simulink model "Shaddad_NavFusion"  (R2026b)
undefined symbols (not defined in the file): P, Ts
libraries: simulink x18, robotcorelib x4, ros2lib x3, mspfiltlib x2
(part 1 of 2)
settings Model: Creator=aomar  LastModifiedBy=aomar

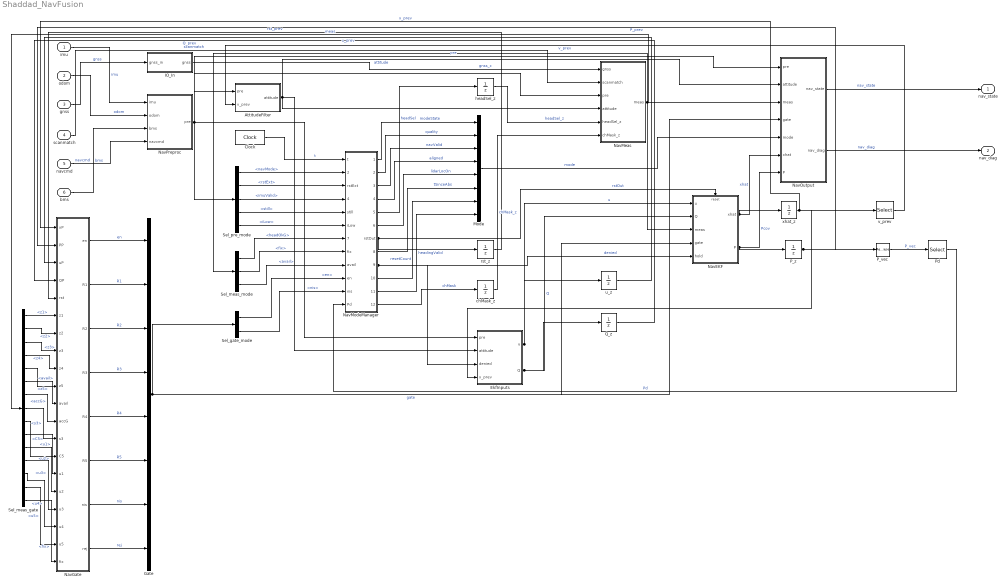
== system Shaddad_NavFusion ==
  imu : Inport  OutDataTypeStr=Bus: Bus_ImuMeas  SampleTime=Ts.imu  BusOutputAsStruct=on
  odom : Inport  Port=2  OutDataTypeStr=Bus: Bus_OdomMeas  SampleTime=Ts.ctrl  BusOutputAsStruct=on
  gnss : Inport  Port=3  OutDataTypeStr=Bus: Bus_GnssRaw  SampleTime=Ts.hk  BusOutputAsStruct=on
  scanmatch : Inport  Port=4  OutDataTypeStr=Bus: Bus_ScanMatchMeas  SampleTime=Ts.gnc_status  BusOutputAsStruct=on
  navcmd : Inport  Port=5  OutDataTypeStr=Bus: Bus_NavCmd  SampleTime=Ts.comm  BusOutputAsStruct=on
  bms : Inport  Port=6  OutDataTypeStr=Bus: Bus_BmsStatus  SampleTime=Ts.hk  BusOutputAsStruct=on
  AttitudeFilter : Subsystem
  Clock : DigitalClock  SampleTime=Ts.nav
  EkfInputs : Subsystem
  Gate : BusCreator  Inputs=8
  IO_In : Subsystem  Variant=on
  Mode : BusCreator  Inputs=8
  NavEKF : Subsystem  Description=EKF (MATLAB System sens_nav_ekf = extendedKalmanFilter, predict + 5 gated corrections at 0.01 s) inside a Resettable Subsystem: navReset rising edge / FAULT re-initialise x0 / P0 (T-NAV-09).  TreatAsAtomicUnit=on
  NavGate : MATLAB Function  TreatAsAtomicUnit=on  mask{prm=P.sensors.navgate}
  NavMeas : Subsystem
  NavModeManager : MATLAB Function  TreatAsAtomicUnit=on  mask{prm=P.sensors.navmode}
  NavOutput : Subsystem
  NavPreproc : Subsystem
  P_vec : Reshape
  P_z : UnitDelay  InitialCondition=P.sensors.ekf.P0  SampleTime=Ts.nav
  Pd : Selector  InputPortWidth=121  IndexOptions=Index vector (dialog)  Indices=[1 13 37]  OutputSizes=1
  Q_z : UnitDelay  InitialCondition=P.sensors.ekf.Qd  SampleTime=Ts.nav
  Sel_gate_mode : BusSelector  OutputSignals=en,nis
  Sel_meas_gate : BusSelector  OutputSignals=z1,z2,z3,z4,z5,avail,accG,s3,C5,u1,u2,u3,u4,u5,fix
  Sel_meas_mode : BusSelector  OutputSignals=headOkG,fix,avail
  Sel_pre_mode : BusSelector  OutputSignals=navMode,rstExt,imuValid,still,iLow
  chMask_z : UnitDelay  InitialCondition=true(5, 1)  SampleTime=Ts.nav
  headSel_z : UnitDelay  SampleTime=Ts.nav
  rst_z : UnitDelay  InitialCondition=false  SampleTime=Ts.nav
  u_z : UnitDelay  InitialCondition=P.sensors.ekf.u0  SampleTime=Ts.nav
  v_prev : Selector  InputPortWidth=11  IndexOptions=Index vector (dialog)  Indices=5  OutputSizes=1
  xhat_z : UnitDelay  InitialCondition=P.sensors.ekf.x0  SampleTime=Ts.nav
  nav_state : Outport  OutDataTypeStr=Bus: Bus_NavState  SampleTime=Ts.ctrl  BusOutputAsStruct=on
  nav_diag : Outport  Port=2  OutDataTypeStr=Bus: Bus_NavDiag  SampleTime=Ts.ctrl  BusOutputAsStruct=on
  wires:
  Sel_meas_gate/1 -> NavGate/6(z1)  "<z1>"
  Sel_meas_gate/2 -> NavGate/7(z2)  "<z2>"
  Sel_meas_gate/3 -> NavGate/8(z3)  "<z3>"
  Sel_meas_gate/4 -> NavGate/9(z4)  "<z4>"
  Sel_meas_gate/5 -> NavGate/10(z5)  "<z5>"
  Sel_meas_gate/6 -> NavGate/11(avail)  "<avail>"
  Sel_meas_gate/8 -> NavGate/13(s3)  "<s3>"
  Sel_meas_gate/10 -> NavGate/15(u1)  "<u1>"
  Sel_meas_gate/12 -> NavGate/17(u3)  "<u3>"
  Sel_meas_gate/14 -> NavGate/19(u5)  "<u5>"
  Sel_meas_gate/15 -> NavGate/20(fix)  "<fix>"
  imu/1 -> NavPreproc/1(imu)  "imu"
  odom/1 -> NavPreproc/2(odom)  "odom"
  gnss/1 -> IO_In/1(gnss_in)  "gnss"
  scanmatch/1 -> NavMeas/2(scanmatch)  "scanmatch"
  navcmd/1 -> NavPreproc/4(navcmd)  "navcmd"
  bms/1 -> NavPreproc/3(bms)  "bms"
  NavGate/1(en) -> Gate/1  "en"
  NavGate/2(R1) -> Gate/2  "R1"
  NavGate/3(R2) -> Gate/3  "R2"
  NavGate/4(R3) -> Gate/4  "R3"
  NavGate/5(R4) -> Gate/5  "R4"
  NavGate/6(R5) -> Gate/6  "R5"
  NavGate/7(nis) -> Gate/7  "nis"
  NavGate/8(rej) -> Gate/8  "rej"
  Gate/1 -> NavOutput/4(gate), NavEKF/4(gate), Sel_gate_mode/1  "gate"
  IO_In/1(gnss) -> NavMeas/1(gnss)  "gnss_c"
  NavPreproc/1(pre) -> EkfInputs/1(pre), Sel_pre_mode/1, NavOutput/1(pre), AttitudeFilter/1(pre), NavMeas/3(pre)  "pre"
  Sel_pre_mode/1 -> NavModeManager/2(navMode)  "<navMode>"
  Sel_pre_mode/2 -> NavModeManager/3(rstExt)  "<rstExt>"
  Sel_pre_mode/3 -> NavModeManager/4(imuValid)  "<imuValid>"
  Sel_pre_mode/4 -> NavModeManager/5(still)  "<still>"
  Sel_pre_mode/5 -> NavModeManager/6(iLow)  "<iLow>"
  Sel_meas_mode/1 -> NavModeManager/7(headOkG)  "<headOkG>"
  Sel_meas_mode/2 -> NavModeManager/8(fix)  "<fix>"
  Sel_meas_mode/3 -> NavModeManager/9(avail)  "<avail>"
  Sel_gate_mode/1 -> NavModeManager/10(en)  "<en>"
  Sel_gate_mode/2 -> NavModeManager/11(nis)  "<nis>"
  Clock/1 -> NavModeManager/1(t)  "t"
  AttitudeFilter/1(attitude) -> EkfInputs/2(attitude), NavOutput/2(attitude), NavMeas/4(attitude)  "attitude"
  NavModeManager/1(modeState) -> Mode/1  "modeState"
  NavModeManager/2(quality) -> Mode/2  "quality"
  NavModeManager/3(navValid) -> Mode/3  "navValid"
  NavModeManager/4(aligned) -> Mode/4  "aligned"
  NavModeManager/5(headSel) -> headSel_z/1  "headSel"
  NavModeManager/6(lidarLocOn) -> Mode/5  "lidarLocOn"
  NavModeManager/7(rstOut) -> NavEKF/Reset, rst_z/1  "rstOut"
  NavModeManager/8(tSinceAbs) -> Mode/6  "tSinceAbs"
  NavModeManager/9(denied) -> EkfInputs/3(denied), NavEKF/5(hold)  "denied"
  NavModeManager/10(resetCount) -> Mode/7  "resetCount"
  NavModeManager/11(headingValid) -> Mode/8  "headingValid"
  NavModeManager/12(chMask) -> chMask_z/1  "chMask"
  Mode/1 -> NavOutput/5(mode)  "mode"
  headSel_z/1 -> NavMeas/5(headSel_z)  "headSel_z"
  rst_z/1 -> NavGate/5(rst)  "rst_prev"
  chMask_z/1 -> NavMeas/6(chMask_z)  "chMask_z"
  EkfInputs/1(u) -> NavEKF/1(u), u_z/1  "u"
  EkfInputs/2(Q) -> NavEKF/2(Q), Q_z/1  "Q"
  u_z/1 -> NavGate/3(uP)  "u_prev"
  NavEKF/1(xhat) -> NavOutput/6(xhat), xhat_z/1  "xhat"
  NavEKF/2(P) -> NavOutput/7(P), P_z/1  "Pcov"
  xhat_z/1 -> EkfInputs/4(x_prev), NavGate/1(xP), v_prev/1  "x_prev"
  P_z/1 -> NavGate/2(PP), P_vec/1  "P_prev"
  NavOutput/1(nav_state) -> nav_state/1  "nav_state"
  NavOutput/2(nav_diag) -> nav_diag/1  "nav_diag"
  P_vec/1 -> Pd/1  "P_vec"
  v_prev/1 -> AttitudeFilter/2(v_prev)  "v_prev"
  Pd/1 -> NavModeManager/12(Pd)  "Pd"
  Q_z/1 -> NavGate/4(QP)  "Q_prev"
  NavMeas/1(meas) -> Sel_meas_gate/1, Sel_meas_mode/1, NavEKF/3(meas), NavOutput/3(meas)  "meas"
  Sel_meas_gate/11 -> NavGate/16(u2)  "<u2>"
  Sel_meas_gate/13 -> NavGate/18(u4)  "<u4>"
  Sel_meas_gate/7 -> NavGate/12(accG)  "<accG>"
  Sel_meas_gate/9 -> NavGate/14(C5)  "<C5>"

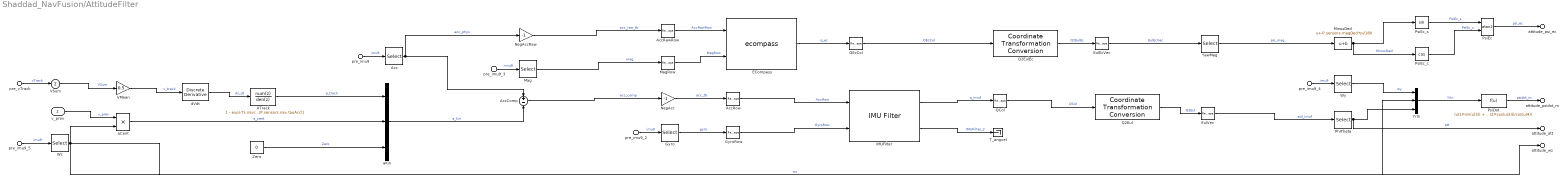
== system Shaddad_NavFusion/AttitudeFilter ==
  pre_imu9 : Inport  PortName=pre  Element=imu9
  pre_imu9_{2..5} (4 alike) : Inport  PortName=pre  Element=imu9
  pre_vTrack : Inport  PortName=pre  Element=vTrack
  v_prev : Inport  Port=2
  ATrack : DiscreteTransferFcn  Numerator=1 - exp(-Ts.nav/P.sensors.nav.tauAcc)  Denominator=[1 -exp(-Ts.nav/P.sensors.nav.tauAcc)]  SampleTime=Ts.nav
  Acc : Selector  InputPortWidth=9  IndexOptions=Index vector (dialog)  Indices=1:3  OutputSizes=1
  AccComp : Sum  Inputs=+-
  AccRawRow : Reshape  OutputDimensionality=Customize  OutputDimensions=[1 3]
  AccRow : Reshape  OutputDimensionality=Customize  OutputDimensions=[1 3]
  ECompass : mspfiltlib/ecompass  ReferenceFrame=ENU  OrientationFormat=quaternion  SimulateUsing=Code generation
  EulEcVec : Reshape
  EulVec : Reshape
  Gyro : Selector  InputPortWidth=9  IndexOptions=Index vector (dialog)  Indices=4:6  OutputSizes=1
  GyroRow : Reshape  OutputDimensionality=Customize  OutputDimensions=[1 3]
  IMUFilter : mspfiltlib/IMU Filter  DispRefFrame=ENU  OrientationFormat=quaternion  DecimationFactor=1  InitialProcessNoise=P.sensors.nav.imufQ0  AccelerometerNoise=P.sensors.imuf.AccelerometerNoise  GyroscopeNoise=P.sensors.imuf.GyroscopeNoise  GyroscopeDriftNoise=P.sensors.imuf.GyroscopeDriftNoise  LinearAccelerationNoise=P.sensors.imuf.LinearAccelerationNoise  LinearAccelerationDecayFactor=P.sensors.imuf.LinearAccelerationDecayFactor  SimulateUsing=Code generation
  Mag : Selector  InputPortWidth=9  IndexOptions=Index vector (dialog)  Indices=7:9  OutputSizes=1
  MagRow : Reshape  OutputDimensionality=Customize  OutputDimensions=[1 3]
  MinusDecl : Bias  Bias=-P.sensors.magDecl*pi/180  SaturateOnIntegerOverflow=off
  NegAcc : Gain  Gain=-1
  NegAccRaw : Gain  Gain=-1
  PhiTheta : Selector  InputPortWidth=3  IndexOptions=Index vector (dialog)  Indices=[3 2]  OutputSizes=1
  PsiDot : Fcn  Expr=(u(1)*sin(u(3)) + u(2)*cos(u(3)))/cos(u(4))
  PsiEc : Trigonometry  Operator=atan2
  PsiEc_c : Trigonometry  Operator=cos
  PsiEc_s : Trigonometry
  Q2Eul : robotcorelib/Coordinate Transformation Conversion  InputRepresentation=Quaternion  InputEulerSequence=ZYX  ShowTrVecInputPort=on  OutputRepresentation=Euler Angles  OutputEulerSequence=ZYX  ShowTrVecOutputPort=on  SimulateUsing=Interpreted execution
      settings: LibrarySourceBlock=navlib/Utilities/Coordinate Transformation Conversion
  Q2EulEc : robotcorelib/Coordinate Transformation Conversion  InputRepresentation=Quaternion  InputEulerSequence=ZYX  ShowTrVecInputPort=on  OutputRepresentation=Euler Angles  OutputEulerSequence=ZYX  ShowTrVecOutputPort=on  SimulateUsing=Interpreted execution
      settings: LibrarySourceBlock=navlib/Utilities/Coordinate Transformation Conversion
  QCol : Reshape  OutputDimensionality=Column vector (2-D)
  QEcCol : Reshape  OutputDimensionality=Column vector (2-D)
  T_angvel : Terminator
  VMean : Gain  Gain=0.5
  VSum : Sum  Inputs=+
  Wy : Selector  InputPortWidth=9  IndexOptions=Index vector (dialog)  Indices=5  OutputSizes=1
  Wz : Selector  InputPortWidth=9  IndexOptions=Index vector (dialog)  Indices=6  OutputSizes=1
  YawMag : Selector  InputPortWidth=3  IndexOptions=Index vector (dialog)  Indices=1  OutputSizes=1
  YrIn : Concatenate  NumInputs=3
  Zero : Constant  Value=0
  aCent : Product
  aKin : Concatenate  NumInputs=3
  dVdt : simulink/Discrete/Discrete Derivative  gainval=1  ICPrevScaledInput=0  OutMin=[]  OutMax=[]  OutDataType=fixdt(1, 16)  OutScaling=2^-10  DoSatur=off
  attitude_att : Outport  PortName=attitude  Element=att
  attitude_psi_ec : Outport  PortName=attitude  Element=psi_ec
  attitude_psidot_m : Outport  PortName=attitude  Element=psidot_m
  attitude_wz : Outport  PortName=attitude  Element=wz
  wires:
  pre_vTrack/1 -> VSum/1  "vTrack"
  pre_imu9_5/1 -> Wz/1  "imu9"
  VSum/1 -> VMean/1  "VSum"
  v_prev/1 -> aCent/1  "v_prev"
  Wz/1 -> YrIn/2, aCent/2, attitude_wz/1  "wz"
  VMean/1 -> dVdt/1  "v_track"
  aCent/1 -> aKin/2  "a_cent"
  dVdt/1 -> ATrack/1  "dv_dt"
  Zero/1 -> aKin/3  "Zero"
  ATrack/1 -> aKin/1  "a_track"
  pre_imu9/1 -> Acc/1  "imu9"
  aKin/1 -> AccComp/2  "a_kin"
  Acc/1 -> AccComp/1, NegAccRaw/1  "acc_phys"
  pre_imu9_3/1 -> Mag/1  "imu9"
  AccComp/1 -> NegAcc/1  "acc_comp"
  NegAccRaw/1 -> AccRawRow/1  "acc_raw_tb"
  Mag/1 -> MagRow/1  "mag"
  pre_imu9_2/1 -> Gyro/1  "imu9"
  AccRawRow/1 -> ECompass/1  "AccRawRow"
  MagRow/1 -> ECompass/2  "MagRow"
  NegAcc/1 -> AccRow/1  "acc_tb"
  Gyro/1 -> GyroRow/1  "gyro"
  AccRow/1 -> IMUFilter/1  "AccRow"
  GyroRow/1 -> IMUFilter/2  "GyroRow"
  ECompass/1 -> QEcCol/1  "q_ec"
  QEcCol/1 -> Q2EulEc/1  "QEcCol"
  IMUFilter/1 -> QCol/1  "q_imuf"
  IMUFilter/2 -> T_angvel/1  "IMUFilter_2"
  QCol/1 -> Q2Eul/1  "QCol"
  Q2EulEc/1 -> EulEcVec/1  "Q2EulEc"
  EulEcVec/1 -> YawMag/1  "EulEcVec"
  Q2Eul/1 -> EulVec/1  "Q2Eul"
  EulVec/1 -> PhiTheta/1  "eul_imuf"
  YawMag/1 -> MinusDecl/1  "psi_mag"
  pre_imu9_4/1 -> Wy/1  "imu9"
  MinusDecl/1 -> PsiEc_s/1, PsiEc_c/1  "MinusDecl"
  Wy/1 -> YrIn/1  "wy"
  PhiTheta/1 -> YrIn/3, attitude_att/1  "att"
  YrIn/1 -> PsiDot/1  "YrIn"
  PsiEc_s/1 -> PsiEc/1  "PsiEc_s"
  PsiEc_c/1 -> PsiEc/2  "PsiEc_c"
  PsiEc/1 -> attitude_psi_ec/1  "psi_ec"
  PsiDot/1 -> attitude_psidot_m/1  "psidot_m"

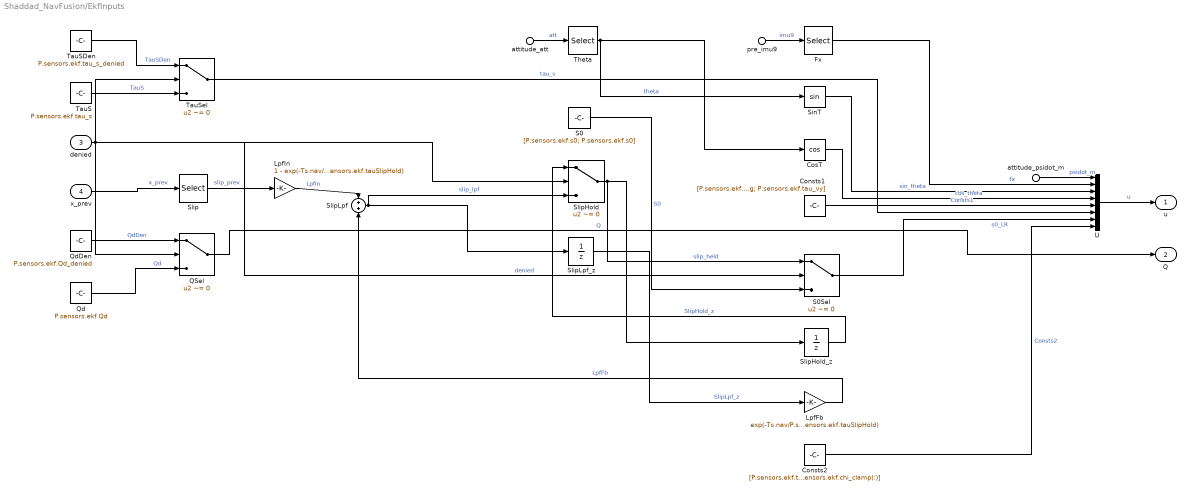
== system Shaddad_NavFusion/EkfInputs ==
  pre_imu9 : Inport  PortName=pre  Element=imu9
  attitude_att : Inport  Port=2  PortName=attitude  Element=att
  attitude_psidot_m : Inport  Port=2  PortName=attitude  Element=psidot_m
  denied : Inport  Port=3
  x_prev : Inport  Port=4
  Consts1 : Constant  Value=[P.sensors.ekf.Ts; P.sensors.g; P.sensors.ekf.tau_vy]
  Consts2 : Constant  Value=[P.sensors.ekf.tau_chi; P.sensors.ekf.chi0; P.sensors.ekf.slip_clamp(:); P.sensors.ekf.chi_clamp(:)]
  CosT : Trigonometry  Operator=cos
  Fx : Selector  InputPortWidth=9  IndexOptions=Index vector (dialog)  Indices=1  OutputSizes=1
  LpfFb : Gain  Gain=exp(-Ts.nav/P.sensors.ekf.tauSlipHold)
  LpfIn : Gain  Gain=1 - exp(-Ts.nav/P.sensors.ekf.tauSlipHold)
  QSel : Switch  Criteria=u2 ~= 0  SaturateOnIntegerOverflow=off  InputSameDT=off
  Qd : Constant  Value=P.sensors.ekf.Qd
  QdDen : Constant  Value=P.sensors.ekf.Qd_denied
  S0 : Constant  Value=[P.sensors.ekf.s0; P.sensors.ekf.s0]
  S0Sel : Switch  Criteria=u2 ~= 0  SaturateOnIntegerOverflow=off  InputSameDT=off
  SinT : Trigonometry
  Slip : Selector  InputPortWidth=11  IndexOptions=Index vector (dialog)  Indices=9:10  OutputSizes=1
  SlipHold : Switch  Criteria=u2 ~= 0  SaturateOnIntegerOverflow=off  InputSameDT=off
  SlipHold_z : UnitDelay  InitialCondition=[P.sensors.ekf.s0; P.sensors.ekf.s0]  SampleTime=Ts.nav
  SlipLpf : Sum
  SlipLpf_z : UnitDelay  InitialCondition=[P.sensors.ekf.s0; P.sensors.ekf.s0]  SampleTime=Ts.nav
  TauS : Constant  Value=P.sensors.ekf.tau_s
  TauSDen : Constant  Value=P.sensors.ekf.tau_s_denied
  TauSel : Switch  Criteria=u2 ~= 0  SaturateOnIntegerOverflow=off  InputSameDT=off
  Theta : Selector  InputPortWidth=2  IndexOptions=Index vector (dialog)  Indices=2  OutputSizes=1
  U : Concatenate  NumInputs=8
  u : Outport
  Q : Outport  Port=2
  wires:
  TauSDen/1 -> TauSel/1  "TauSDen"
  TauS/1 -> TauSel/3  "TauS"
  denied/1 -> S0Sel/2, QSel/2, TauSel/2, SlipHold/2  "denied"
  x_prev/1 -> Slip/1  "x_prev"
  QdDen/1 -> QSel/1  "QdDen"
  Qd/1 -> QSel/3  "Qd"
  Slip/1 -> LpfIn/1  "slip_prev"
  TauSel/1 -> U/6  "tau_s"
  QSel/1 -> Q/1  "Q"
  LpfIn/1 -> SlipLpf/1  "LpfIn"
  SlipLpf/1 -> SlipLpf_z/1, SlipHold/3  "slip_lpf"
  attitude_att/1 -> Theta/1  "att"
  S0/1 -> S0Sel/3  "S0"
  SlipLpf_z/1 -> LpfFb/1  "SlipLpf_z"
  Theta/1 -> CosT/1, SinT/1  "theta"
  SlipHold/1 -> SlipHold_z/1, S0Sel/1  "slip_held"
  pre_imu9/1 -> Fx/1  "imu9"
  SinT/1 -> U/3  "sin_theta"
  CosT/1 -> U/4  "cos_theta"
  Consts1/1 -> U/5  "Consts1"
  LpfFb/1 -> SlipLpf/2  "LpfFb"
  Consts2/1 -> U/8  "Consts2"
  SlipHold_z/1 -> SlipHold/1  "SlipHold_z"
  Fx/1 -> U/2  "fx"
  S0Sel/1 -> U/7  "s0_LR"
  attitude_psidot_m/1 -> U/1  "psidot_m"
  U/1 -> u/1  "u"

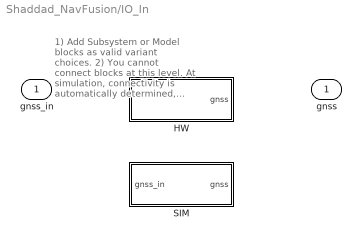
== system Shaddad_NavFusion/IO_In ==
  note: 1) Add Subsystem or Model blocks as valid variant choices.
      | 2) You cannot connect blocks at this level. At simulation, connectivity is automatically
      | determined, based on the active variant and port name matching.
  gnss_in : Inport
  HW : Subsystem  Description=sens_acq_gnss (T12, HW choice of Shaddad_NavFusion/IO_In, VC_TARGET == 1; 0.1 s). Ports: out 1 gnss Bus_GnssRaw 0.1. ros2lib/Subscribe (At sample time) of the ROS 2 ublox driver standard topics: /fix sensor_msgs/NavSatFix (t_meas = header.stamp, lla, hAcc / vAcc = sqrt(position_covariance(1 / 9)), fixType from status: -1 -> 0, 0 / 1 -> 1, 2 -> 4 if hAcc < rtkFixedAcc else 5; newData = IsNew), /fix_velocity geometry_msgs/TwistWithCovarianceStamped (vel_ENU, sAcc), /navheading sensor_msgs/Imu (baseline yaw ENU -> heading_deg = mod(90 - yaw, 360), headAcc_deg, headingValid = IsNew and headAcc < headAccMax_deg). numSV and corrAge are not carried by the standard messages (0). Parameters P.sensors.acq_gnss.  VariantControl=VC_TARGET == 1
  SIM : Subsystem  VariantControl=VC_TARGET == 0
  gnss : Outport

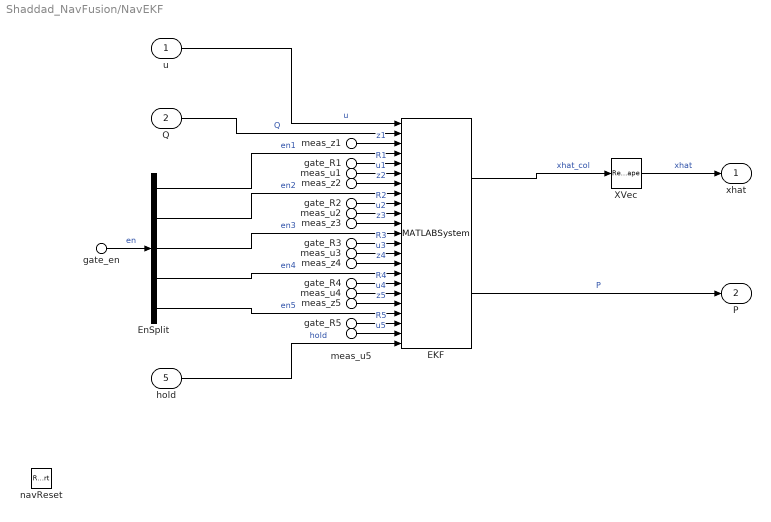
== system Shaddad_NavFusion/NavEKF ==
  u : Inport
  Q : Inport  Port=2
  meas_z1 : Inport  Port=3  PortName=meas  Element=z1
  meas_u1 : Inport  Port=3  PortName=meas  Element=u1
  meas_z2 : Inport  Port=3  PortName=meas  Element=z2
  meas_u2 : Inport  Port=3  PortName=meas  Element=u2
  meas_z3 : Inport  Port=3  PortName=meas  Element=z3
  meas_u3 : Inport  Port=3  PortName=meas  Element=u3
  meas_z4 : Inport  Port=3  PortName=meas  Element=z4
  meas_u4 : Inport  Port=3  PortName=meas  Element=u4
  meas_z5 : Inport  Port=3  PortName=meas  Element=z5
  meas_u5 : Inport  Port=3  PortName=meas  Element=u5
  gate_en : Inport  Port=4  PortName=gate  Element=en
  gate_R1 : Inport  Port=4  PortName=gate  Element=R1
  gate_R2 : Inport  Port=4  PortName=gate  Element=R2
  gate_R3 : Inport  Port=4  PortName=gate  Element=R3
  gate_R4 : Inport  Port=4  PortName=gate  Element=R4
  gate_R5 : Inport  Port=4  PortName=gate  Element=R5
  hold : Inport  Port=5
  navReset : ResetPort  DisableCoverage=on
  EKF : MATLABSystem  System=sens_nav_ekf  InitialState=P.sensors.ekf.x0  InitialStateCovariance=P.sensors.ekf.P0
      mask Type: sens_nav_ekf
  EnSplit : Demux  Outputs=5
  XVec : Reshape
  xhat : Outport
  P : Outport  Port=2
  wires:
  gate_en/1 -> EnSplit/1  "en"
  EnSplit/1 -> EKF/4  "en1"
  EnSplit/2 -> EKF/8  "en2"
  EnSplit/3 -> EKF/12  "en3"
  EnSplit/4 -> EKF/16  "en4"
  EnSplit/5 -> EKF/20  "en5"
  u/1 -> EKF/1  "u"
  Q/1 -> EKF/2  "Q"
  hold/1 -> EKF/23  "hold"
  meas_z1/1 -> EKF/3  "z1"
  gate_R1/1 -> EKF/5  "R1"
  meas_u1/1 -> EKF/6  "u1"
  meas_z2/1 -> EKF/7  "z2"
  gate_R2/1 -> EKF/9  "R2"
  meas_u2/1 -> EKF/10  "u2"
  meas_z3/1 -> EKF/11  "z3"
  gate_R3/1 -> EKF/13  "R3"
  meas_u3/1 -> EKF/14  "u3"
  meas_z4/1 -> EKF/15  "z4"
  gate_R4/1 -> EKF/17  "R4"
  meas_u4/1 -> EKF/18  "u4"
  meas_z5/1 -> EKF/19  "z5"
  gate_R5/1 -> EKF/21  "R5"
  meas_u5/1 -> EKF/22  "u5"
  EKF/1 -> XVec/1  "xhat_col"
  EKF/2 -> P/1  "P"
  XVec/1 -> xhat/1  "xhat"

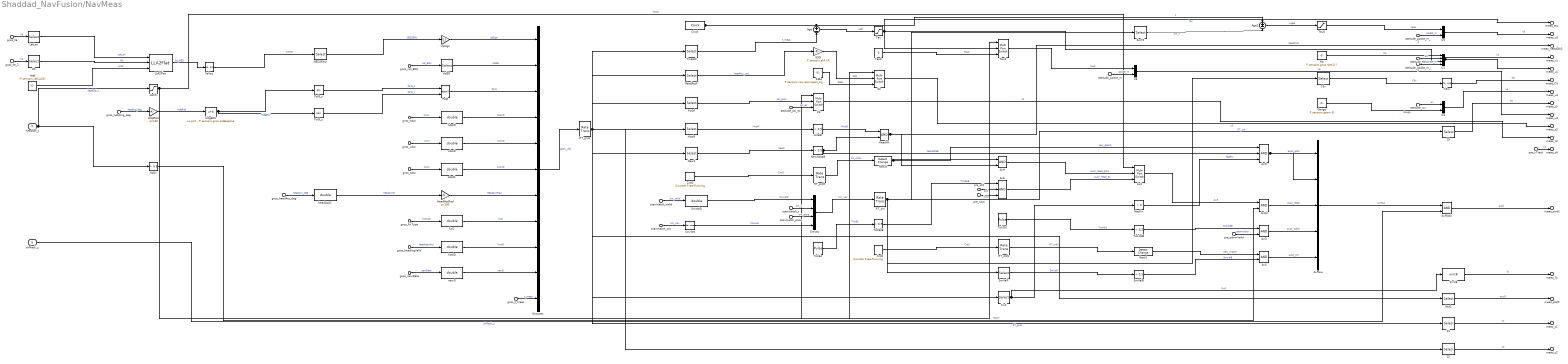
== system Shaddad_NavFusion/NavMeas ==
  gnss_lla : Inport  PortName=gnss  Element=lla
  gnss_lla_2 : Inport  PortName=gnss  Element=lla
  gnss_vel_ENU : Inport  PortName=gnss  Element=vel_ENU
  gnss_heading_deg : Inport  PortName=gnss  Element=heading_deg
  gnss_hAcc : Inport  PortName=gnss  Element=hAcc
  gnss_vAcc : Inport  PortName=gnss  Element=vAcc
  gnss_sAcc : Inport  PortName=gnss  Element=sAcc
  gnss_headAcc_deg : Inport  PortName=gnss  Element=headAcc_deg
  gnss_fixType : Inport  PortName=gnss  Element=fixType
  gnss_headingValid : Inport  PortName=gnss  Element=headingValid
  gnss_newData : Inport  PortName=gnss  Element=newData
  gnss_t_meas : Inport  PortName=gnss  Element=t_meas
  scanmatch_valid : Inport  Port=2  PortName=scanmatch  Element=valid
  scanmatch_cov : Inport  Port=2  PortName=scanmatch  Element=cov
  scanmatch_t : Inport  Port=2  PortName=scanmatch  Element=t
  scanmatch_pose : Inport  Port=2  PortName=scanmatch  Element=pose
  pre_still : Inport  Port=3  PortName=pre  Element=still
  pre_iLow : Inport  Port=3  PortName=pre  Element=iLow
  pre_odomValid : Inport  Port=3  PortName=pre  Element=odomValid
  pre_vTrack : Inport  Port=3  PortName=pre  Element=vTrack
  attitude_psi_ec : Inport  Port=4  PortName=attitude  Element=psi_ec
  attitude_psidot_m : Inport  Port=4  PortName=attitude  Element=psidot_m
  attitude_psidot_m_2 : Inport  Port=4  PortName=attitude  Element=psidot_m
  attitude_psidot_m_3 : Inport  Port=4  PortName=attitude  Element=psidot_m
  attitude_wz : Inport  Port=4  PortName=attitude  Element=wz
  attitude_att : Inport  Port=4  PortName=attitude  Element=att
  headSel_z : Inport  Port=5
  chMask_z : Inport  Port=6
  AccG : Selector  InputPortWidth=14  IndexOptions=Index vector (dialog)  Indices=7:9  OutputSizes=1
  Age : Sum  Inputs=+-
  AgeS : Sum  Inputs=+-
  Alt : Selector  InputPortWidth=3  IndexOptions=Index vector (dialog)  Indices=3  OutputSizes=1
  Av3 : MultiPortSwitch  Inputs=2  SaturateOnIntegerOverflow=off  InputSameDT=off
  AvE : Logic  Inputs=3  AllPortsSameDT=off  OutDataTypeStr=boolean
  AvG : Logic  Inputs=3  AllPortsSameDT=off  OutDataTypeStr=boolean
  AvH : Logic  AllPortsSameDT=off  OutDataTypeStr=boolean
  AvHd : Logic  AllPortsSameDT=off  OutDataTypeStr=boolean
  AvMask : Logic  AllPortsSameDT=off  OutDataTypeStr=boolean
  AvO : Logic  AllPortsSameDT=off  OutDataTypeStr=boolean
  AvRaw : Concatenate  NumInputs=5
  AvS : Logic  AllPortsSameDT=off  OutDataTypeStr=boolean
  C5m : Reshape  OutputDimensionality=Customize  OutputDimensions=[3 3]
  C5v : Selector  InputPortWidth=14  IndexOptions=Index vector (dialog)  Indices=6:14  OutputSizes=1
  Clock : DigitalClock  SampleTime=Ts.nav
  CntG : simulink/Sources/Counter Free-Running  NumBits=16  tsamp=Ts.gnss
  CntS : simulink/Sources/Counter Free-Running  NumBits=16  tsamp=Ts.scanmatch
  CovVec : Reshape
  FixF : Selector  InputPortWidth=14  IndexOptions=Index vector (dialog)  Indices=11  OutputSizes=1
  FixU8 : DataTypeConversion  OutDataTypeStr=uint8  RndMeth=Floor
  Gauge : Constant  Value=P.sensors.geom.B
  GnssVec : Concatenate  NumInputs=11
  HValB : simulink/Logic and Bit Operations/Compare To Constant  relop=>  const=0.5  OutDataTypeStr=boolean
  HValF : Selector  InputPortWidth=14  IndexOptions=Index vector (dialog)  Indices=12  OutputSizes=1
  HasFix : simulink/Logic and Bit Operations/Compare To Constant  relop=>  const=0  OutDataTypeStr=boolean
  HdgENU : Bias  Bias=pi/2 - P.sensors.gnss.psiBaseline  SaturateOnIntegerOverflow=off
  HdgRad : Gain  Gain=-pi/180
  HeadAccF : Selector  InputPortWidth=14  IndexOptions=Index vector (dialog)  Indices=10  OutputSizes=1
  HeadAccRad : Gain  Gain=pi/180
  HeadOk : Logic  AllPortsSameDT=off  OutDataTypeStr=boolean
  Href : Constant  Value=-P.sensors.refLLA(3)
  HsCtl : Saturate  UpperLimit=2  LowerLimit=1
  HsOn : simulink/Logic and Bit Operations/Compare To Constant  relop=>  const=0.5  OutDataTypeStr=boolean
  LLA2Flat : LLA2Flat  LL0=P.sensors.refLLA(1:2)
  LatLon : Selector  InputPortWidth=3  IndexOptions=Index vector (dialog)  Indices=[1 2]  OutputSizes=1
  NED2ENU : Selector  InputPortWidth=3  IndexOptions=Index vector (dialog)  Indices=[2 1 3]  OutputSizes=1
  NewDataB : simulink/Logic and Bit Operations/Compare To Constant  relop=>  const=0.5  OutDataTypeStr=boolean
  NewF : Selector  InputPortWidth=14  IndexOptions=Index vector (dialog)  Indices=13  OutputSizes=1
  NewG : simulink/Logic and Bit Operations/Detect Change  vinit=0  OutDataTypeStr=boolean
  NewS : simulink/Logic and Bit Operations/Detect Change  vinit=0  OutDataTypeStr=boolean
  PsiG : Trigonometry  Operator=atan2
  PsiG_c : Trigonometry  Operator=cos
  PsiG_s : Trigonometry
  PsiGf : Selector  InputPortWidth=14  IndexOptions=Index vector (dialog)  Indices=6  OutputSizes=1
  RT_cntG : RateTransition  OutPortSampleTime=Ts.nav
  RT_cntS : RateTransition  OutPortSampleTime=Ts.nav
  RT_gnss : RateTransition  OutPortSampleTime=Ts.nav
  RT_sm : RateTransition  OutPortSampleTime=Ts.nav
  Ra : Constant  Value=P.sensors.gnss.rAnt1(:)
  S3 : MultiPortSwitch  Inputs=2  SaturateOnIntegerOverflow=off  InputSameDT=off
  S3Ec : Constant  Value=P.sensors.nav.ecompass_sig
  S3G : Gain  Gain=P.sensors.ekf.kR
  SmTF : Selector  InputPortWidth=14  IndexOptions=Index vector (dialog)  Indices=2  OutputSizes=1
  SmValB : simulink/Logic and Bit Operations/Compare To Constant  relop=>  const=0.5  OutDataTypeStr=boolean
  SmValD : DataTypeConversion  OutDataTypeStr=double  RndMeth=Floor
  SmValF : Selector  InputPortWidth=14  IndexOptions=Index vector (dialog)  Indices=1  OutputSizes=1
  SmVec : Concatenate  NumInputs=4
  Tau : Saturate  UpperLimit=P.sensors.nav.tauMax  LowerLimit=0
  Tau0 : Constant  Value=0
  Tau3 : MultiPortSwitch  Inputs=2  SaturateOnIntegerOverflow=off  InputSameDT=off
  Tau5 : Saturate  UpperLimit=P.sensors.nav.tauMaxSm  LowerLimit=0
  TickEc : DiscretePulseGenerator  Period=P.sensors.ekf.headDecim  SampleTime=Ts.nav
  TickEcB : simulink/Logic and Bit Operations/Compare To Constant  relop=>  const=0.5  OutDataTypeStr=boolean
  TickOd : DiscretePulseGenerator  Period=P.sensors.ekf.odomDecim  PhaseDelay=2  SampleTime=Ts.nav
  TickOdB : simulink/Logic and Bit Operations/Compare To Constant  relop=>  const=0.5  OutDataTypeStr=boolean
  TmeasF : Selector  InputPortWidth=14  IndexOptions=Index vector (dialog)  Indices=14  OutputSizes=1
  U1 : Concatenate  NumInputs=4
  U3 : Concatenate
  U4 : Concatenate
  U5 : Concatenate
  UpSign : Gain  Gain=[1 1 -1]
  VelEN : Selector  InputPortWidth=3  IndexOptions=Index vector (dialog)  Indices=[1 2]  OutputSizes=1
  XeVec : Reshape
  Z1 : Selector  InputPortWidth=14  IndexOptions=Index vector (dialog)  Indices=1:3  OutputSizes=1
  Z2 : Selector  InputPortWidth=14  IndexOptions=Index vector (dialog)  Indices=4:5  OutputSizes=1
  Z3 : MultiPortSwitch  Inputs=2  SaturateOnIntegerOverflow=off  InputSameDT=off
  Z5 : Selector  InputPortWidth=14  IndexOptions=Index vector (dialog)  Indices=3:5  OutputSizes=1
  fixD : DataTypeConversion  OutDataTypeStr=double  RndMeth=Floor
  hAccD : DataTypeConversion  OutDataTypeStr=double  RndMeth=Floor
  hValD : DataTypeConversion  OutDataTypeStr=double  RndMeth=Floor
  headAccD : DataTypeConversion  OutDataTypeStr=double  RndMeth=Floor
  newD : DataTypeConversion  OutDataTypeStr=double  RndMeth=Floor
  sAccD : DataTypeConversion  OutDataTypeStr=double  RndMeth=Floor
  vAccD : DataTypeConversion  OutDataTypeStr=double  RndMeth=Floor
  meas_z1 : Outport  PortName=meas  Element=z1
  meas_z2 : Outport  PortName=meas  Element=z2
  meas_accG : Outport  PortName=meas  Element=accG
  meas_fix : Outport  PortName=meas  Element=fix
  meas_tau : Outport  PortName=meas  Element=tau
  meas_headOkG : Outport  PortName=meas  Element=headOkG
  meas_z3 : Outport  PortName=meas  Element=z3
  meas_s3 : Outport  PortName=meas  Element=s3
  meas_u3 : Outport  PortName=meas  Element=u3
  meas_z4 : Outport  PortName=meas  Element=z4
  meas_u4 : Outport  PortName=meas  Element=u4
  meas_u5 : Outport  PortName=meas  Element=u5
  meas_C5 : Outport  PortName=meas  Element=C5
  meas_z5 : Outport  PortName=meas  Element=z5
  meas_avail : Outport  PortName=meas  Element=avail
  meas_u1 : Outport  PortName=meas  Element=u1
  meas_u2 : Outport  PortName=meas  Element=u2
  wires:
  gnss_lla/1 -> LatLon/1  "lla"
  gnss_lla_2/1 -> Alt/1  "lla"
  Href/1 -> LLA2Flat/3  "Href"
  headSel_z/1 -> HsOn/1, HsCtl/1  "headSel_z"
  chMask_z/1 -> AvMask/2  "chMask_z"
  LatLon/1 -> LLA2Flat/1  "LatLon"
  Alt/1 -> LLA2Flat/2  "Alt"
  gnss_heading_deg/1 -> HdgRad/1  "heading_deg"
  HsCtl/1 -> Av3/1, Tau3/1, S3/1, Z3/1  "HsCtl"
  HdgRad/1 -> HdgENU/1  "HdgRad"
  HsOn/1 -> AvHd/2  "HsOn"
  LLA2Flat/1 -> XeVec/1  "Xe_NED"
  XeVec/1 -> NED2ENU/1  "XeVec"
  HdgENU/1 -> PsiG_s/1, PsiG_c/1  "HdgENU"
  gnss_headAcc_deg/1 -> headAccD/1  "headAcc_deg"
  PsiG_s/1 -> PsiG/1  "PsiG_s"
  PsiG_c/1 -> PsiG/2  "PsiG_c"
  NED2ENU/1 -> UpSign/1  "NED2ENU"
  headAccD/1 -> HeadAccRad/1  "headAccD"
  gnss_vel_ENU/1 -> VelEN/1  "vel_ENU"
  gnss_hAcc/1 -> hAccD/1  "hAcc"
  gnss_vAcc/1 -> vAccD/1  "vAcc"
  gnss_sAcc/1 -> sAccD/1  "sAcc"
  gnss_fixType/1 -> fixD/1  "fixType"
  gnss_headingValid/1 -> hValD/1  "headingValid"
  gnss_newData/1 -> newD/1  "newData"
  UpSign/1 -> GnssVec/1  "UpSign"
  PsiG/1 -> GnssVec/3  "PsiG"
  HeadAccRad/1 -> GnssVec/7  "HeadAccRad"
  VelEN/1 -> GnssVec/2  "VelEN"
  hAccD/1 -> GnssVec/4  "hAccD"
  vAccD/1 -> GnssVec/5  "vAccD"
  sAccD/1 -> GnssVec/6  "sAccD"
  fixD/1 -> GnssVec/8  "fixD"
  hValD/1 -> GnssVec/9  "hValD"
  newD/1 -> GnssVec/10  "newD"
  gnss_t_meas/1 -> GnssVec/11  "t_meas"
  GnssVec/1 -> RT_gnss/1  "gnss_vec"
  RT_gnss/1 -> Z2/1, Z1/1, AccG/1, FixF/1, TmeasF/1, HeadAccF/1, PsiGf/1, NewF/1, HValF/1  "RT_gnss"
  scanmatch_valid/1 -> SmValD/1  "sm_valid"
  scanmatch_cov/1 -> CovVec/1  "sm_cov"
  CntG/1 -> RT_cntG/1  "CntG"
  CovVec/1 -> SmVec/4  "CovVec"
  TmeasF/1 -> Age/2  "t_meas"
  HeadAccF/1 -> S3G/1  "headAcc_rad"
  PsiGf/1 -> Z3/2  "psi_gnss"
  HValF/1 -> HValB/1  "HValF"
  NewF/1 -> NewDataB/1  "NewF"
  Clock/1 -> AgeS/1, Age/1  "t"
  SmValD/1 -> SmVec/1  "SmValD"
  attitude_psi_ec/1 -> Z3/3  "psi_ec"
  scanmatch_t/1 -> SmVec/2  "sm_t"
  scanmatch_pose/1 -> SmVec/3  "sm_pose"
  SmVec/1 -> RT_sm/1  "sm_vec"
  Age/1 -> Tau/1  "Age"
  S3G/1 -> S3/2  "S3G"
  S3Ec/1 -> S3/3  "S3Ec"
  HValB/1 -> HeadOk/1  "HValB"
  NewDataB/1 -> HeadOk/2, AvG/2  "NewDataB"
  TickEc/1 -> TickEcB/1  "TickEc"
  Z3/1 -> meas_z3/1  "z3"
  RT_cntG/1 -> NewG/1  "RT_cntG"
  Tau/1 -> U1/3, Tau3/2, meas_tau/1  "tau"
  Tau0/1 -> Tau3/3  "Tau0"
  TickEcB/1 -> AvE/1  "TickEcB"
  CntS/1 -> RT_cntS/1  "CntS"
  S3/1 -> meas_s3/1  "s3"
  RT_sm/1 -> SmTF/1, C5v/1, SmValF/1, Z5/1  "RT_sm"
  HeadOk/1 -> meas_headOkG/1, AvH/2  "headOkG"
  NewG/1 -> AvG/1, AvH/1  "new_epoch"
  pre_still/1 -> AvE/2  "still"
  pre_iLow/1 -> AvE/3  "iLow"
  AvH/1 -> Av3/2  "avail_head_gnss"
  AvE/1 -> Av3/3  "avail_head_ec"
  TickOd/1 -> TickOdB/1  "TickOd"
  Tau3/1 -> U3/1  "tau3"
  RT_cntS/1 -> NewS/1  "RT_cntS"
  SmValF/1 -> SmValB/1  "SmValF"
  FixF/1 -> HasFix/1, FixU8/1  "FixF"
  attitude_psidot_m/1 -> U3/2  "psidot_m"
  U3/1 -> meas_u3/1  "u3"
  HasFix/1 -> AvG/3  "HasFix"
  TickOdB/1 -> AvO/1  "TickOdB"
  SmValB/1 -> AvS/2  "SmValB"
  Av3/1 -> AvHd/1  "Av3"
  SmTF/1 -> AgeS/2  "sm_t"
  NewS/1 -> AvS/1  "new_match"
  pre_odomValid/1 -> AvO/2  "odomValid"
  AgeS/1 -> Tau5/1  "AgeS"
  AvG/1 -> AvRaw/2, AvRaw/1  "avail_gnss"
  AvHd/1 -> AvRaw/3  "avail_head"
  AvO/1 -> AvRaw/4  "avail_odom"
  AvS/1 -> AvRaw/5  "avail_sm"
  AvRaw/1 -> AvMask/1  "AvRaw"
  Tau5/1 -> U5/1  "tau5"
  Ra/1 -> U1/1  "Ra"
  Gauge/1 -> U4/2  "Gauge"
  C5v/1 -> C5m/1  "C5v"
  attitude_psidot_m_2/1 -> U5/2  "psidot_m"
  attitude_att/1 -> U1/2  "att"
  attitude_psidot_m_3/1 -> U1/4  "psidot_m"
  attitude_wz/1 -> U4/1  "wz"
  U5/1 -> meas_u5/1  "u5"
  U1/1 -> meas_u2/1, meas_u1/1  "u1"
  U4/1 -> meas_u4/1  "u4"
  C5m/1 -> meas_C5/1  "C5"
  AvMask/1 -> meas_avail/1  "avail"
  Z5/1 -> meas_z5/1  "z5"
  AccG/1 -> meas_accG/1  "accG"
  Z1/1 -> meas_z1/1  "z1"
  Z2/1 -> meas_z2/1  "z2"
  FixU8/1 -> meas_fix/1  "fix"
  pre_vTrack/1 -> meas_z4/1  "z4"

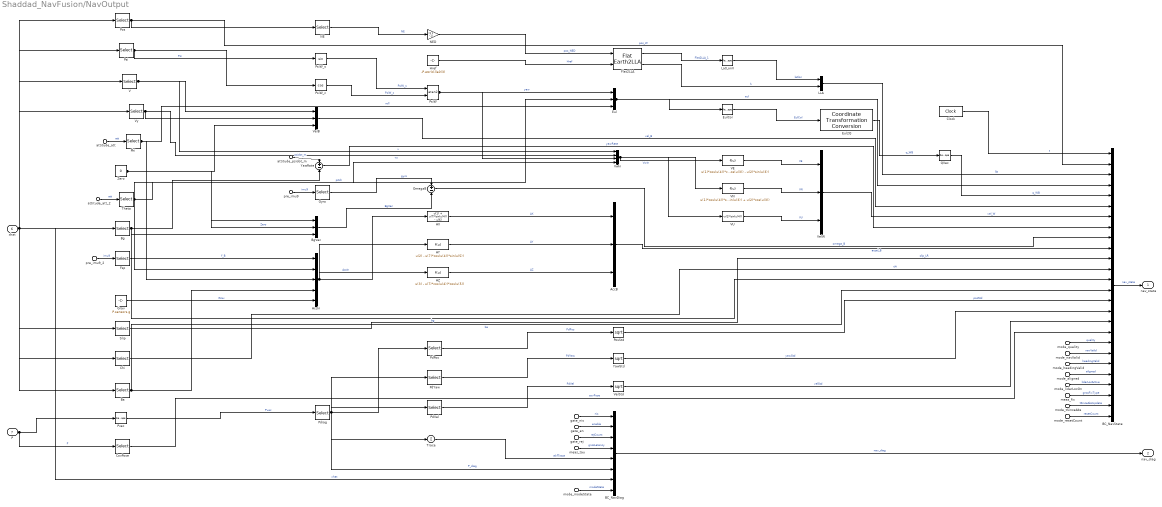
== system Shaddad_NavFusion/NavOutput ==
  pre_imu9 : Inport  PortName=pre  Element=imu9
  pre_imu9_2 : Inport  PortName=pre  Element=imu9
  attitude_att : Inport  Port=2  PortName=attitude  Element=att
  attitude_att_2 : Inport  Port=2  PortName=attitude  Element=att
  attitude_psidot_m : Inport  Port=2  PortName=attitude  Element=psidot_m
  meas_fix : Inport  Port=3  PortName=meas  Element=fix
  meas_tau : Inport  Port=3  PortName=meas  Element=tau
  gate_nis : Inport  Port=4  PortName=gate  Element=nis
  gate_en : Inport  Port=4  PortName=gate  Element=en
  gate_rej : Inport  Port=4  PortName=gate  Element=rej
  mode_quality : Inport  Port=5  PortName=mode  Element=quality
  mode_navValid : Inport  Port=5  PortName=mode  Element=navValid
  mode_headingValid : Inport  Port=5  PortName=mode  Element=headingValid
  mode_aligned : Inport  Port=5  PortName=mode  Element=aligned
  mode_lidarLocOn : Inport  Port=5  PortName=mode  Element=lidarLocOn
  mode_tSinceAbs : Inport  Port=5  PortName=mode  Element=tSinceAbs
  mode_resetCount : Inport  Port=5  PortName=mode  Element=resetCount
  mode_modeState : Inport  Port=5  PortName=mode  Element=modeState
  xhat : Inport  Port=6
  P : Inport  Port=7
  AX : Fcn  Expr=u(1) + u(7)*sin(u(4)) - u(6)
  AY : Fcn  Expr=u(2) - u(7)*cos(u(4))*sin(u(5))
  AZ : Fcn  Expr=u(3) - u(7)*cos(u(4))*cos(u(5))
  AccB : Concatenate  NumInputs=3
  AccIn : Concatenate  NumInputs=5
  BC_NavDiag : BusCreator  Inputs=8  OutDataTypeStr=Bus: Bus_NavDiag  NonVirtualBus=on
      settings: InheritFromInputs=off
  BC_NavState : BusCreator  Inputs=26  OutDataTypeStr=Bus: Bus_NavState  NonVirtualBus=on
      settings: InheritFromInputs=off
  Ba : Selector  InputPortWidth=11  IndexOptions=Index vector (dialog)  Indices=8  OutputSizes=1
  Bg : Selector  InputPortWidth=11  IndexOptions=Index vector (dialog)  Indices=7  OutputSizes=1
  BgVec : Concatenate  NumInputs=3
  Chi : Selector  InputPortWidth=11  IndexOptions=Index vector (dialog)  Indices=11  OutputSizes=1
  Clock : DigitalClock  SampleTime=Ts.nav
  CovPose : Selector  NumberOfDimensions=2  InputPortWidth=3  IndexOptions=Index vector (dialog),Index vector (dialog)  Indices=[1 2 4],[1 2 4]  OutputSizes=1
  Eul : Concatenate  NumInputs=3
  Eul2Q : robotcorelib/Coordinate Transformation Conversion  InputRepresentation=Euler Angles  InputEulerSequence=ZYX  ShowTrVecInputPort=on  OutputRepresentation=Quaternion  OutputEulerSequence=ZYX  ShowTrVecOutputPort=on  SimulateUsing=Interpreted execution
      settings: LibrarySourceBlock=navlib/Utilities/Coordinate Transformation Conversion
  EulCol : Reshape  OutputDimensionality=Column vector (2-D)
  Flat2LLA : FlatEarth2LLA  LL0=P.sensors.refLLA(1:2)
  Fsp : Selector  InputPortWidth=9  IndexOptions=Index vector (dialog)  Indices=1:3  OutputSizes=1
  Grav : Constant  Value=P.sensors.g
  Gyro : Selector  InputPortWidth=9  IndexOptions=Index vector (dialog)  Indices=4:6  OutputSizes=1
  Href : Constant  Value=-P.world.lla0(3)
  LLA : Concatenate
  LatLonV : Reshape
  NE : Selector  InputPortWidth=3  IndexOptions=Index vector (dialog)  Indices=[2 1 3]  OutputSizes=1
  NED : Gain  Gain=[1 1 -1]
  OmegaB : Sum  Inputs=+-
  PdPos : Selector  InputPortWidth=11  IndexOptions=Index vector (dialog)  Indices=1:3  OutputSizes=1
  PdVel : Selector  InputPortWidth=11  IndexOptions=Index vector (dialog)  Indices=5  OutputSizes=1
  PdYaw : Selector  InputPortWidth=11  IndexOptions=Index vector (dialog)  Indices=4  OutputSizes=1
  Pdiag : Selector  InputPortWidth=121  IndexOptions=Index vector (dialog)  Indices=1:12:121  OutputSizes=1
  Phi : Selector  InputPortWidth=2  IndexOptions=Index vector (dialog)  Indices=1  OutputSizes=1
  Pos : Selector  InputPortWidth=11  IndexOptions=Index vector (dialog)  Indices=1:3  OutputSizes=1
  PosStd : Math  Operator=sqrt
  Psi : Selector  InputPortWidth=11  IndexOptions=Index vector (dialog)  Indices=4  OutputSizes=1
  PsiW : Trigonometry  Operator=atan2
  PsiW_c : Trigonometry  Operator=cos
  PsiW_s : Trigonometry
  Pvec : Reshape
  QVec : Reshape
  Slip : Selector  InputPortWidth=11  IndexOptions=Index vector (dialog)  Indices=9:10  OutputSizes=1
  Theta : Selector  InputPortWidth=2  IndexOptions=Index vector (dialog)  Indices=2  OutputSizes=1
  Trace : Sum  Inputs=+
  V : Selector  InputPortWidth=11  IndexOptions=Index vector (dialog)  Indices=5  OutputSizes=1
  VE : Fcn  Expr=u(1)*cos(u(4))*cos(u(3)) - u(2)*sin(u(3))
  VN : Fcn  Expr=u(1)*cos(u(4))*sin(u(3)) + u(2)*cos(u(3))
  VU : Fcn  Expr=-u(1)*sin(u(4))
  VelB : Concatenate  NumInputs=3
  VelStd : Math  Operator=sqrt
  VelW : Concatenate  NumInputs=3
  VwIn : Concatenate  NumInputs=4
  Vy : Selector  InputPortWidth=11  IndexOptions=Index vector (dialog)  Indices=6  OutputSizes=1
  YawRate : Sum  Inputs=+-
  YawStd : Math  Operator=sqrt
  Zero : Constant  Value=0
  nav_state : Outport
  nav_diag : Outport  Port=2
  wires:
  xhat/1 -> BC_NavDiag/7, Pos/1, Psi/1, Ba/1, V/1, Chi/1, Vy/1, Slip/1, Bg/1  "xhat"
  P/1 -> Pvec/1, CovPose/1  "P"
  pre_imu9_2/1 -> Fsp/1  "imu9"
  attitude_att_2/1 -> Theta/1  "att"
  attitude_att/1 -> Phi/1  "att"
  Zero/1 -> BgVec/2, BgVec/1, VelB/3  "Zero"
  Grav/1 -> AccIn/5  "Grav"
  Pvec/1 -> Pdiag/1  "Pvec"
  Pos/1 -> BC_NavState/2, NE/1  "pos_W"
  Bg/1 -> YawRate/2, BC_NavState/13, BgVec/3  "bg"
  Fsp/1 -> AccIn/1  "f_B"
  Slip/1 -> BC_NavState/11  "slip_LR"
  Chi/1 -> BC_NavState/12  "chi"
  Ba/1 -> AccIn/4, BC_NavState/14  "ba"
  CovPose/1 -> BC_NavState/18  "covPose"
  Psi/1 -> PsiW_c/1, PsiW_s/1  "Psi"
  Theta/1 -> Eul/2, AccIn/2, VwIn/4  "pitch"
  V/1 -> VwIn/1, VelB/1  "v"
  Phi/1 -> AccIn/3, Eul/3  "roll"
  Vy/1 -> VwIn/2, VelB/2  "vy"
  attitude_psidot_m/1 -> YawRate/1  "psidot_m"
  pre_imu9/1 -> Gyro/1  "imu9"
  VelB/1 -> BC_NavState/6  "vel_B"
  BgVec/1 -> OmegaB/2  "BgVec"
  AccIn/1 -> AX/1, AY/1, AZ/1  "AccIn"
  YawRate/1 -> BC_NavState/8  "yawRate"
  PsiW_s/1 -> PsiW/1  "PsiW_s"
  PsiW_c/1 -> PsiW/2  "PsiW_c"
  NE/1 -> NED/1  "NE"
  Gyro/1 -> OmegaB/1  "gyro"
  Pdiag/1 -> PdPos/1, BC_NavDiag/6, PdYaw/1, Trace/1, PdVel/1  "P_diag"
  OmegaB/1 -> BC_NavState/9  "omega_B"
  Trace/1 -> BC_NavDiag/5  "ekfTrace"
  NED/1 -> Flat2LLA/1  "pos_NED"
  Href/1 -> Flat2LLA/2  "Href"
  PsiW/1 -> VwIn/3, Eul/1  "yaw"
  PdPos/1 -> PosStd/1  "PdPos"
  PdYaw/1 -> YawStd/1  "PdYaw"
  PdVel/1 -> VelStd/1  "PdVel"
  AX/1 -> AccB/1  "AX"
  AY/1 -> AccB/2  "AY"
  AZ/1 -> AccB/3  "AZ"
  gate_nis/1 -> BC_NavDiag/1  "nis"
  gate_en/1 -> BC_NavDiag/2  "enable"
  gate_rej/1 -> BC_NavDiag/3  "rejCount"
  meas_tau/1 -> BC_NavDiag/4  "gnssLatency"
  mode_modeState/1 -> BC_NavDiag/8  "modeState"
  Eul/1 -> BC_NavState/4, EulCol/1  "eul"
  AccB/1 -> BC_NavState/10  "accel_B"
  BC_NavDiag/1 -> nav_diag/1  "nav_diag"
  VwIn/1 -> VU/1, VN/1, VE/1  "VwIn"
  PosStd/1 -> BC_NavState/15  "posStd"
  YawStd/1 -> BC_NavState/16  "yawStd"
  VelStd/1 -> BC_NavState/17  "velStd"
  Flat2LLA/1 -> LatLonV/1  "Flat2LLA_1"
  Flat2LLA/2 -> LLA/2  "h"
  LatLonV/1 -> LLA/1  "latlon"
  EulCol/1 -> Eul2Q/1  "EulCol"
  VE/1 -> VelW/1  "VE"
  VN/1 -> VelW/2  "VN"
  VU/1 -> VelW/3  "VU"
  LLA/1 -> BC_NavState/3  "lla"
  VelW/1 -> BC_NavState/7  "vel_W"
  Eul2Q/1 -> QVec/1  "q_WB"
  QVec/1 -> BC_NavState/5  "q_WB"
  Clock/1 -> BC_NavState/1  "t"
  mode_quality/1 -> BC_NavState/19  "quality"
  mode_navValid/1 -> BC_NavState/20  "navValid"
  mode_headingValid/1 -> BC_NavState/21  "headingValid"
  mode_aligned/1 -> BC_NavState/22  "aligned"
  mode_lidarLocOn/1 -> BC_NavState/23  "lidarLocActive"
  meas_fix/1 -> BC_NavState/24  "gnssFixType"
  mode_tSinceAbs/1 -> BC_NavState/25  "tSinceAbsUpdate"
  mode_resetCount/1 -> BC_NavState/26  "resetCount"
  BC_NavState/1 -> nav_state/1  "nav_state"

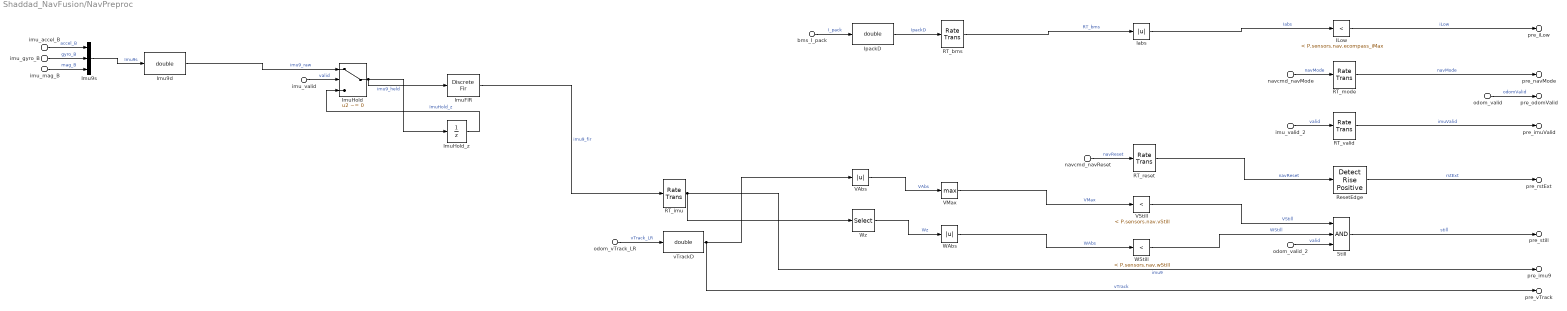
== system Shaddad_NavFusion/NavPreproc ==
  imu_accel_B : Inport  PortName=imu  Element=accel_B
  imu_gyro_B : Inport  PortName=imu  Element=gyro_B
  imu_mag_B : Inport  PortName=imu  Element=mag_B
  imu_valid : Inport  PortName=imu  Element=valid
  imu_valid_2 : Inport  PortName=imu  Element=valid
  odom_vTrack_LR : Inport  Port=2  PortName=odom  Element=vTrack_LR
  odom_valid : Inport  Port=2  PortName=odom  Element=valid
  odom_valid_2 : Inport  Port=2  PortName=odom  Element=valid
  bms_I_pack : Inport  Port=3  PortName=bms  Element=I_pack
  navcmd_navMode : Inport  Port=4  PortName=navcmd  Element=navMode
  navcmd_navReset : Inport  Port=4  PortName=navcmd  Element=navReset
  ILow : simulink/Logic and Bit Operations/Compare To Constant  relop=<  const=P.sensors.nav.ecompass_iMax  OutDataTypeStr=boolean
  Iabs : Abs  SaturateOnIntegerOverflow=off
  Imu9d : DataTypeConversion  OutDataTypeStr=double  RndMeth=Floor
  Imu9s : Concatenate  NumInputs=3
  ImuFIR : DiscreteFir  SampleTime=Ts.imu
  ImuHold : Switch  Criteria=u2 ~= 0  SaturateOnIntegerOverflow=off  InputSameDT=off
  ImuHold_z : UnitDelay  InitialCondition=[0; 0; P.sensors.g; 0; 0; 0; 0; 0; 0]  SampleTime=Ts.imu
  IpackD : DataTypeConversion  OutDataTypeStr=double  RndMeth=Floor
  RT_bms : RateTransition  OutPortSampleTime=Ts.nav
  RT_imu : RateTransition  OutPortSampleTime=Ts.nav
  RT_mode : RateTransition  OutPortSampleTime=Ts.nav
  RT_reset : RateTransition  OutPortSampleTime=Ts.nav
  RT_valid : RateTransition  OutPortSampleTime=Ts.nav
  ResetEdge : simulink/Logic and Bit Operations/Detect Rise Positive  vinit=0  OutDataTypeStr=boolean
  Still : Logic  Inputs=3  AllPortsSameDT=off  OutDataTypeStr=boolean
  VAbs : Abs  SaturateOnIntegerOverflow=off
  VMax : MinMax  Function=max
  VStill : simulink/Logic and Bit Operations/Compare To Constant  relop=<  const=P.sensors.nav.vStill  OutDataTypeStr=boolean
  WAbs : Abs  SaturateOnIntegerOverflow=off
  WStill : simulink/Logic and Bit Operations/Compare To Constant  relop=<  const=P.sensors.nav.wStill  OutDataTypeStr=boolean
  Wz : Selector  InputPortWidth=9  IndexOptions=Index vector (dialog)  Indices=6  OutputSizes=1
  vTrackD : DataTypeConversion  OutDataTypeStr=double  RndMeth=Floor
  pre_imu9 : Outport  PortName=pre  Element=imu9
  pre_imuValid : Outport  PortName=pre  Element=imuValid
  pre_vTrack : Outport  PortName=pre  Element=vTrack
  pre_odomValid : Outport  PortName=pre  Element=odomValid
  pre_iLow : Outport  PortName=pre  Element=iLow
  pre_navMode : Outport  PortName=pre  Element=navMode
  pre_rstExt : Outport  PortName=pre  Element=rstExt
  pre_still : Outport  PortName=pre  Element=still
  wires:
  imu_accel_B/1 -> Imu9s/1  "accel_B"
  imu_gyro_B/1 -> Imu9s/2  "gyro_B"
  imu_mag_B/1 -> Imu9s/3  "mag_B"
  Imu9s/1 -> Imu9d/1  "Imu9s"
  Imu9d/1 -> ImuHold/1  "imu9_raw"
  imu_valid/1 -> ImuHold/2  "valid"
  ImuHold/1 -> ImuHold_z/1, ImuFIR/1  "imu9_held"
  ImuHold_z/1 -> ImuHold/3  "ImuHold_z"
  ImuFIR/1 -> RT_imu/1  "imu9_fir"
  odom_vTrack_LR/1 -> vTrackD/1  "vTrack_LR"
  RT_imu/1 -> pre_imu9/1, Wz/1  "imu9"
  vTrackD/1 -> VAbs/1, pre_vTrack/1  "vTrack"
  bms_I_pack/1 -> IpackD/1  "I_pack"
  VAbs/1 -> VMax/1  "VAbs"
  Wz/1 -> WAbs/1  "Wz"
  IpackD/1 -> RT_bms/1  "IpackD"
  VMax/1 -> VStill/1  "VMax"
  WAbs/1 -> WStill/1  "WAbs"
  RT_bms/1 -> Iabs/1  "RT_bms"
  navcmd_navReset/1 -> RT_reset/1  "navReset"
  Iabs/1 -> ILow/1  "Iabs"
  VStill/1 -> Still/1  "VStill"
  WStill/1 -> Still/2  "WStill"
  RT_reset/1 -> ResetEdge/1  "navReset"
  navcmd_navMode/1 -> RT_mode/1  "navMode"
  imu_valid_2/1 -> RT_valid/1  "valid"
  odom_valid_2/1 -> Still/3  "valid"
  ILow/1 -> pre_iLow/1  "iLow"
  Still/1 -> pre_still/1  "still"
  RT_mode/1 -> pre_navMode/1  "navMode"
  RT_valid/1 -> pre_imuValid/1  "imuValid"
  ResetEdge/1 -> pre_rstExt/1  "rstExt"
  odom_valid/1 -> pre_odomValid/1  "odomValid"

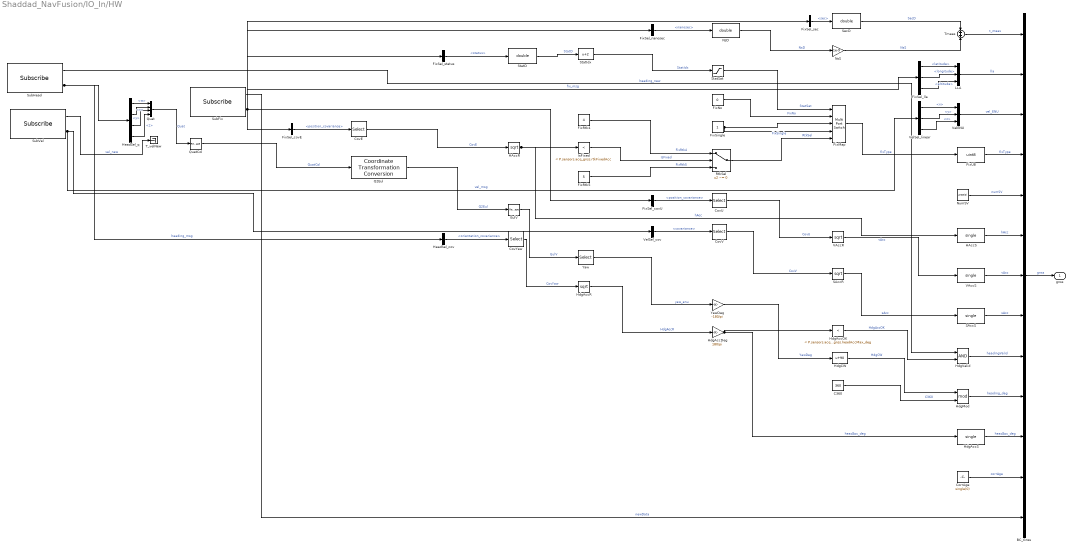
== system Shaddad_NavFusion/IO_In/HW ==
  BC_Gnss : BusCreator  Inputs=13  OutDataTypeStr=Bus: Bus_GnssRaw  NonVirtualBus=on
      settings: InheritFromInputs=off
  C360 : Constant  Value=360
  CorrAge : Constant  Value=single(0)  OutDataTypeStr=single
  CovE : Selector  InputPortWidth=9  IndexOptions=Index vector (dialog)  Indices=1  OutputSizes=1
  CovU : Selector  InputPortWidth=9  IndexOptions=Index vector (dialog)  Indices=9  OutputSizes=1
  CovV : Selector  InputPortWidth=36  IndexOptions=Index vector (dialog)  Indices=1  OutputSizes=1
  CovYaw : Selector  InputPortWidth=9  IndexOptions=Index vector (dialog)  Indices=9  OutputSizes=1
  EulV : Reshape
  FixMap : MultiPortSwitch  Inputs=4  SaturateOnIntegerOverflow=off  InputSameDT=off
  FixNo : Constant  Value=0
  FixRtk4 : Constant  Value=4
  FixRtk5 : Constant  Value=5
  FixSel_covE : BusSelector  OutputSignals=position_covariance
  FixSel_covU : BusSelector  OutputSignals=position_covariance
  FixSel_lla : BusSelector  OutputSignals=latitude,longitude,altitude
  FixSel_nanosec : BusSelector  OutputSignals=header.stamp.nanosec
  FixSel_sec : BusSelector  OutputSignals=header.stamp.sec
  FixSel_status : BusSelector  OutputSignals=status.status
  FixSingle : Constant
  FixU8 : DataTypeConversion  OutDataTypeStr=uint8  RndMeth=Floor
  HAccR : Math  Operator=sqrt
  HAccS : DataTypeConversion  OutDataTypeStr=single  RndMeth=Floor
  HdgAccDeg : Gain  Gain=180/pi
  HdgAccOK : simulink/Logic and Bit Operations/Compare To Constant  relop=<  const=P.sensors.acq_gnss.headAccMax_deg  OutDataTypeStr=boolean
  HdgAccR : Math  Operator=sqrt
  HdgAccS : DataTypeConversion  OutDataTypeStr=single  RndMeth=Floor
  HdgCW : Bias  Bias=90  SaturateOnIntegerOverflow=off
  HdgMod : Math  Operator=mod
  HdgValid : Logic  AllPortsSameDT=off  OutDataTypeStr=boolean
  HeadSel_cov : BusSelector  OutputSignals=orientation_covariance
  HeadSel_q : BusSelector  OutputSignals=orientation.w,orientation.x,orientation.y,orientation.z
  IsFixed : simulink/Logic and Bit Operations/Compare To Constant  relop=<  const=P.sensors.acq_gnss.rtkFixedAcc  OutDataTypeStr=boolean
  LLA : Concatenate  NumInputs=3
  NsD : DataTypeConversion  OutDataTypeStr=double  RndMeth=Floor
  NsS : Gain  Gain=1e-9
  NumSV : Constant  Value=uint8(0)  OutDataTypeStr=uint8
  Q2Eul : robotcorelib/Coordinate Transformation Conversion  InputRepresentation=Quaternion  InputEulerSequence=ZYX  ShowTrVecInputPort=on  OutputRepresentation=Euler Angles  OutputEulerSequence=ZYX  ShowTrVecOutputPort=on  SimulateUsing=Interpreted execution
      settings: LibrarySourceBlock=navlib/Utilities/Coordinate Transformation Conversion
  Quat : Concatenate  NumInputs=4
  QuatCol : Reshape  OutputDimensionality=Column vector (2-D)
  RtkSel : Switch  Criteria=u2 ~= 0  SaturateOnIntegerOverflow=off  InputSameDT=off
  SAccR : Math  Operator=sqrt
  SAccS : DataTypeConversion  OutDataTypeStr=single  RndMeth=Floor
  SecD : DataTypeConversion  OutDataTypeStr=double  RndMeth=Floor
  StatD : DataTypeConversion  OutDataTypeStr=double  RndMeth=Floor
  StatIdx : Bias  Bias=2  SaturateOnIntegerOverflow=off
  StatSat : Saturate  UpperLimit=4  LowerLimit=1
  SubFix : ros2lib/Subscribe  topicSource=Specify your own  topic=/fix  messageType=sensor_msgs/NavSatFix  SubscriberMode=At sample time  sampleTime=P.sensors.acq_gnss.Ts  CallbackGroupType=Default  CallbackGroupName=callback_group_1  QOSHistory=Keep last  QOSDepth=10  QOSReliability=Reliable  QOSDurability=Volatile  QOSDeadline=Inf  QOSLifespan=Inf  QOSLiveliness=Automatic  QOSLeaseDuration=Inf  QOSAvoidROSNamespaceConventions=off
  SubHead : ros2lib/Subscribe  topicSource=Specify your own  topic=/navheading  messageType=sensor_msgs/Imu  SubscriberMode=At sample time  sampleTime=P.sensors.acq_gnss.Ts  CallbackGroupType=Default  CallbackGroupName=callback_group_1  QOSHistory=Keep last  QOSDepth=10  QOSReliability=Reliable  QOSDurability=Volatile  QOSDeadline=Inf  QOSLifespan=Inf  QOSLiveliness=Automatic  QOSLeaseDuration=Inf  QOSAvoidROSNamespaceConventions=off
  SubVel : ros2lib/Subscribe  topicSource=Specify your own  topic=/fix_velocity  messageType=geometry_msgs/TwistWithCovarianceStamped  SubscriberMode=At sample time  sampleTime=P.sensors.acq_gnss.Ts  CallbackGroupType=Default  CallbackGroupName=callback_group_1  QOSHistory=Keep last  QOSDepth=10  QOSReliability=Reliable  QOSDurability=Volatile  QOSDeadline=Inf  QOSLifespan=Inf  QOSLiveliness=Automatic  QOSLeaseDuration=Inf  QOSAvoidROSNamespaceConventions=off
  T_velNew : Terminator
  Tmeas : Sum
  VAccR : Math  Operator=sqrt
  VAccS : DataTypeConversion  OutDataTypeStr=single  RndMeth=Floor
  VelENU : Concatenate  NumInputs=3
  VelSel_cov : BusSelector  OutputSignals=twist.covariance
  VelSel_linear : BusSelector  OutputSignals=twist.twist.linear.x,twist.twist.linear.y,twist.twist.linear.z
  Yaw : Selector  InputPortWidth=3  IndexOptions=Index vector (dialog)  Indices=1  OutputSizes=1
  YawDeg : Gain  Gain=-180/pi
  gnss : Outport  OutDataTypeStr=Bus: Bus_GnssRaw
  wires:
  SubHead/1 -> HdgValid/1  "heading_new"
  SubHead/2 -> HeadSel_cov/1, HeadSel_q/1  "heading_msg"
  SubVel/1 -> T_velNew/1  "vel_new"
  SubVel/2 -> VelSel_cov/1, VelSel_linear/1  "vel_msg"
  HeadSel_q/1 -> Quat/1  "<w>"
  HeadSel_q/2 -> Quat/2  "<x>"
  HeadSel_q/3 -> Quat/3  "<y>"
  HeadSel_q/4 -> Quat/4  "<z>"
  Quat/1 -> QuatCol/1  "Quat"
  QuatCol/1 -> Q2Eul/1  "QuatCol"
  SubFix/1 -> BC_Gnss/13  "newData"
  SubFix/2 -> FixSel_covU/1, FixSel_sec/1, FixSel_nanosec/1, FixSel_status/1, FixSel_lla/1, FixSel_covE/1  "fix_msg"
  FixSel_covE/1 -> CovE/1  "<position_covariance>"
  CovE/1 -> HAccR/1  "CovE"
  Q2Eul/1 -> EulV/1  "Q2Eul"
  FixSel_status/1 -> StatD/1  "<status>"
  HeadSel_cov/1 -> CovYaw/1  "<orientation_covariance>"
  HAccR/1 -> HAccS/1, IsFixed/1  "hAcc"
  EulV/1 -> Yaw/1  "EulV"
  CovYaw/1 -> HdgAccR/1  "CovYaw"
  StatD/1 -> StatIdx/1  "StatD"
  FixRtk4/1 -> RtkSel/1  "FixRtk4"
  IsFixed/1 -> RtkSel/2  "IsFixed"
  FixRtk5/1 -> RtkSel/3  "FixRtk5"
  HdgAccR/1 -> HdgAccDeg/1  "HdgAccR"
  StatIdx/1 -> StatSat/1  "StatIdx"
  Yaw/1 -> YawDeg/1  "yaw_enu"
  FixSel_nanosec/1 -> NsD/1  "<nanosec>"
  FixSel_covU/1 -> CovU/1  "<position_covariance>"
  VelSel_cov/1 -> CovV/1  "<covariance>"
  StatSat/1 -> FixMap/1  "StatSat"
  FixNo/1 -> FixMap/2  "FixNo"
  FixSingle/1 -> FixMap/3, FixMap/4  "FixSingle"
  YawDeg/1 -> HdgCW/1  "YawDeg"
  HdgAccDeg/1 -> HdgAccS/1, HdgAccOK/1  "headAcc_deg"
  CovU/1 -> VAccR/1  "CovU"
  CovV/1 -> SAccR/1  "CovV"
  RtkSel/1 -> FixMap/5  "RtkSel"
  NsD/1 -> NsS/1  "NsD"
  FixSel_sec/1 -> SecD/1  "<sec>"
  NsS/1 -> Tmeas/2  "NsS"
  VAccR/1 -> VAccS/1  "vAcc"
  SAccR/1 -> SAccS/1  "sAcc"
  HdgAccOK/1 -> HdgValid/2  "HdgAccOK"
  C360/1 -> HdgMod/2  "C360"
  FixMap/1 -> FixU8/1  "fixType"
  HdgCW/1 -> HdgMod/1  "HdgCW"
  SecD/1 -> Tmeas/1  "SecD"
  FixSel_lla/1 -> LLA/1  "<latitude>"
  FixSel_lla/2 -> LLA/2  "<longitude>"
  FixSel_lla/3 -> LLA/3  "<altitude>"
  VelSel_linear/1 -> VelENU/1  "<x>"
  VelSel_linear/2 -> VelENU/2  "<y>"
  VelSel_linear/3 -> VelENU/3  "<z>"
  LLA/1 -> BC_Gnss/2  "lla"
  VelENU/1 -> BC_Gnss/3  "vel_ENU"
  Tmeas/1 -> BC_Gnss/1  "t_meas"
  NumSV/1 -> BC_Gnss/5  "numSV"
  HdgValid/1 -> BC_Gnss/9  "headingValid"
  HdgMod/1 -> BC_Gnss/10  "heading_deg"
  CorrAge/1 -> BC_Gnss/12  "corrAge"
  FixU8/1 -> BC_Gnss/4  "fixType"
  HAccS/1 -> BC_Gnss/6  "hAcc"
  VAccS/1 -> BC_Gnss/7  "vAcc"
  SAccS/1 -> BC_Gnss/8  "sAcc"
  HdgAccS/1 -> BC_Gnss/11  "headAcc_deg"
  BC_Gnss/1 -> gnss/1  "gnss"

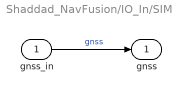
== system Shaddad_NavFusion/IO_In/SIM ==
  gnss_in : Inport
  gnss : Outport
  wires:
  gnss_in/1 -> gnss/1  "gnss"

== matlab function Shaddad_NavFusion/NavModeManager ==
  settings: updateMethod=DISCRETE  sampleTime=Ts.nav  description=Navigation mode manager FSM (subsystems/sensors/sens_nav_mode.m).
  data: t input; modeState output; navMode input; rstExt input; imuValid input; still input; iLow input; headOkG input; fix input; avail input; en input; nis input; Pd input; quality output; navValid output; aligned output; headSel output; lidarLocOn output; rstOut output; tSinceAbs output; denied output; resetCount output; headingValid output; chMask output; prm parameter
function [modeState, quality, navValid, aligned, headSel, lidarLocOn, rstOut, tSinceAbs, denied, resetCount, headingValid, chMask] = fcn(t, navMode, rstExt, imuValid, still, iLow, headOkG, fix, avail, en, nis, Pd, prm)
[modeState, quality, navValid, aligned, headSel, lidarLocOn, rstOut, tSinceAbs, denied, resetCount, headingValid, chMask] = sens_nav_mode(t, navMode, rstExt, imuValid, still, iLow, headOkG, fix, avail, en, nis, Pd, prm);
